simulink model "ZT_VehCtrl_18B_CAN"  (R2018b)
settings: Solver=FixedStepAuto  StartTime=0.0  StopTime=inf  FixedStep=0.005  RelTol=1e-3
InitFcn:
  | mbd_mpc_consistency_checks(bdroot(gcs));
values from neighbouring files (symbols this model uses):
  BatoverTempTh = single(80)    [VCU_INIT.m]
  BRS_PwrValid = single(5)    [VCU_INIT.m]
  BRSEnSpdTh1 = single(10)    [VCU_INIT.m]
  BRSEnSpdTh2 = single(20)    [VCU_INIT.m]
  MCUTempAlarmTh = single (60)    [VCU_INIT.m]
  mps2kmh = single(3.6)    [VCU_INIT.m]
  MtrPwrFac = single(1/9550)    [VCU_INIT.m]
  MtrTempAlarmTh = single (50)    [VCU_INIT.m]
  Padle1Signal1_Th = [PadleSignal1_min,PadleSignal1_max]    [VCU_INIT.m]
  Padle1Signal2_Th = [PadleSignal2_min,PadleSignal2_max]    [VCU_INIT.m]
  PadleSignal1_max = 3.84    [VCU_INIT.m]
  PadleSignal1_min = 0.75    [VCU_INIT.m]
  PadleSignal2_max = 1.92    [VCU_INIT.m]
  PadleSignal2_min = 0.375    [VCU_INIT.m]
  PadleValid = 0.05    [VCU_INIT.m]
  PwrLimFactor = single(0.5)    [VCU_INIT.m]
  Ratio = single(1)    [VCU_INIT.m]
  rpm2mps = single(2*pi/60 * WhlRadius/Ratio)    [VCU_INIT.m]
  SOCLowTh = single(20)    [VCU_INIT.m]
  VehPwrBackwardMax = VehPwrMax * single(0.3)    [VCU_INIT.m]
  VehPwrMax = single(MtrPwrMax * 4)    [VCU_INIT.m]
  VehTrqBackwardMax = VehTrqMax * single(0.3)    [VCU_INIT.m]
  VehTrqMax = single(MtrTrqMax * Ratio *4)    [VCU_INIT.m]
  WhlRadius = single(1)    [VCU_INIT.m]
undefined symbols (not defined in the file or in its folder): Delay_Charge, Delay_Discharge, fifo_0_vect, fifo_1_vect, LQFP, pts1_fifo_0_vect, pts1_fifo_1_vect, pts2_fifo_0_vect, pts2_fifo_1_vect, pts3_fifo_0_vect, pts3_fifo_1_vect, pts4_fifo_0_vect, pts4_fifo_1_vect
libraries: mbd_mpc574x_ec_toolbox x157, canmsglib x74, simulink x38
(part 4 of 12)

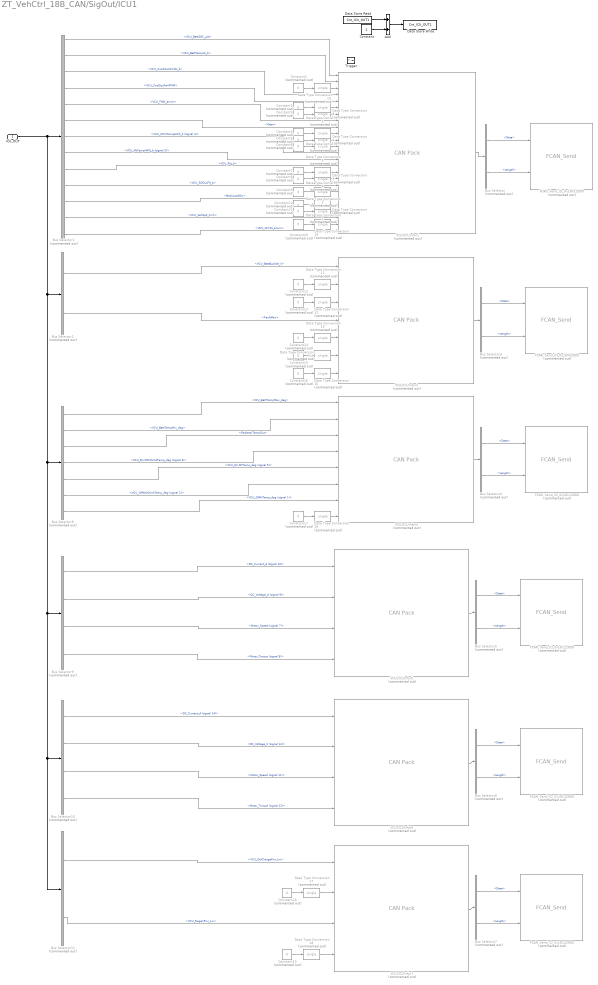
== system ZT_VehCtrl_18B_CAN/SigOut/ICU1  ==
  "ICU_OUT " : Inport
  Trigger : TriggerPort  VariantControl=Variant  PortDimensions=1
  Add : Sum
  Bus Selector{,3..7} (6 alike) : BusSelector  Commented=on  OutputSignals=Data,Length
  Bus Selector1 : BusSelector  Commented=on  OutputSignals=BMS.VCU_BattSOC_pct,BMS.VCU_BattTempHi_b,TMS.VCU_CoolFanWrkIdc_b,TMS.VCU_CoolSysFanPWM,Fault.VCU_FltSt_enum,Gear,MCU.VCU_MCUTempHiFlt_b (signal 4),MCU.VCU_MtTempHiFlt_b (signal 3),signal6.VCU_Pst_b,BMS.VCU_SOCLoFlt_b,signal6.BodyLoadSw,VCU_VehSpd_kmh,VCU_WrkSt_enum
  Bus Selector10 : BusSelector  Commented=on  OutputSignals=MCU.DC_Current_A (signal 14),MCU.DC_Voltage_V (signal 13),MCU.Motor_Speed (signal 11),MCU.Motor_Torque (signal 12)
  Bus Selector11 : BusSelector  Commented=on  OutputSignals=BMS.VCU_DisChargePwr_kw,BMS.VCU_RegenPwr_kw
  Bus Selector2 : BusSelector  Commented=on  OutputSignals=BMS.VCU_BattBusVolt_V,Fault.FaultMax
  Bus Selector8 : BusSelector  Commented=on  OutputSignals=BMS.VCU_BattTempMax_deg,BMS.VCU_BattTempMin_deg,signal6.RadiatorTempOut,MCU.VCU_DrvMtCtlUnitTemp_deg (signal 6),MCU.VCU_DrvMtTemp_deg (signal 5),MCU.VCU_OilMtCtlUnitTemp_deg (signal 2),MCU.VCU_OilMtTemp_deg (signal 1)
  Bus Selector9 : BusSelector  Commented=on  OutputSignals=MCU.DC_Current_A (signal 10),MCU.DC_Voltage_A (signal 9),MCU.Motor_Speed (signal 7),MCU.Motor_Torque (signal 8)
  Constant : Constant  OutDataTypeStr=uint8
  Constant{1..20} (20 alike) : Constant  Commented=on  Value=0  OutDataTypeStr=single
  Data Store Read : DataStoreRead  DataStoreName=Cnt_ICU_OUT1
  Data Store Write : DataStoreWrite  DataStoreName=Cnt_ICU_OUT1
  Data Type Conversion{,1..19} (20 alike) : DataTypeConversion  Commented=on  OutDataTypeStr=single
  FCAN_Send_ID_0x180128D0 : mbd_mpc574x_ec_toolbox/Communication Blocks/CAN Blocks/FCAN_Send  Priority=2  Commented=on  can_instance=0  can_mode=Non-blocking  can_timeout_ms=0  can_mb_idx=16  can_extended_id=on  can_is_remote=off  can_id=180128D0  show_adv_opts=off  can_fd_enable=off  can_enable_brs=off  can_fd_padding=0
      settings: SourceProductName=NXP Model-Based Design Toolbox for MPC57xx MCUs
  FCAN_Send_ID_0x180328D0 : mbd_mpc574x_ec_toolbox/Communication Blocks/CAN Blocks/FCAN_Send  Priority=2  Commented=on  can_instance=0  can_mode=Non-blocking  can_timeout_ms=0  can_mb_idx=18  can_extended_id=on  can_is_remote=off  can_id=180328D0  show_adv_opts=off  can_fd_enable=off  can_enable_brs=off  can_fd_padding=0
      settings: SourceProductName=NXP Model-Based Design Toolbox for MPC57xx MCUs
  FCAN_Send_ID_0x181128D0 : mbd_mpc574x_ec_toolbox/Communication Blocks/CAN Blocks/FCAN_Send  Priority=2  Commented=on  can_instance=0  can_mode=Non-blocking  can_timeout_ms=0  can_mb_idx=19  can_extended_id=on  can_is_remote=off  can_id=181128D0  show_adv_opts=off  can_fd_enable=off  can_enable_brs=off  can_fd_padding=0
      settings: SourceProductName=NXP Model-Based Design Toolbox for MPC57xx MCUs
  FCAN_Send_ID_0x181228D0 : mbd_mpc574x_ec_toolbox/Communication Blocks/CAN Blocks/FCAN_Send  Priority=2  Commented=on  can_instance=0  can_mode=Non-blocking  can_timeout_ms=0  can_mb_idx=20  can_extended_id=on  can_is_remote=off  can_id=181228D0  show_adv_opts=off  can_fd_enable=off  can_enable_brs=off  can_fd_padding=0
      settings: SourceProductName=NXP Model-Based Design Toolbox for MPC57xx MCUs
  FCAN_Send_ID_0x181328D0 : mbd_mpc574x_ec_toolbox/Communication Blocks/CAN Blocks/FCAN_Send  Priority=2  Commented=on  can_instance=0  can_mode=Non-blocking  can_timeout_ms=0  can_mb_idx=21  can_extended_id=on  can_is_remote=off  can_id=181328D0  show_adv_opts=off  can_fd_enable=off  can_enable_brs=off  can_fd_padding=0
      settings: SourceProductName=NXP Model-Based Design Toolbox for MPC57xx MCUs
  FCAN_Send_ID_0x181428D0 : mbd_mpc574x_ec_toolbox/Communication Blocks/CAN Blocks/FCAN_Send  Priority=2  Commented=on  can_instance=0  can_mode=Non-blocking  can_timeout_ms=0  can_mb_idx=22  can_extended_id=on  can_is_remote=off  can_id=181428D0  show_adv_opts=off  can_fd_enable=off  can_enable_brs=off  can_fd_padding=0
      settings: SourceProductName=NXP Model-Based Design Toolbox for MPC57xx MCUs
  VCU2ICUInfor1 : canmsglib/CAN Pack  Commented=on  CANdbFile=D:\VCU\VCU_SL_ZhengZhou\ZT2\模型与接口\CAN_DBC\整车CANA_GBK.dbc  MsgList=(none)  MsgName=VCU2ICUInfor1  MsgIDType=Extended (29-bit identifier)  MsgIdentifier=402729168  MsgLength=8  SignalInfo=VCU_BattSOC_pct$16$8$1$2$1$0$1$0$0$100$#VCU_BattTempHi_b$32$1$1$2$1$0$1$0$0$1$#VCU_BrakeFlt_b$39$1$1$2$1$0$1$0$0$1$#VCU_CoolFanWrkIdc_b$44$1$1$2$1$0$1$0$0$1$#VCU_CoolSysFanPWM$56$8$1$2$1$0$1$0$0$100$#VCU_CoolSysFltIdc_b$43$1$1$2$1$0$1$0$0$1$#VCU_EmrPumpSt_enum$5$2$1$2$1$0$1$0$0$3$#VCU_FltSt_enum$6$1$1$2$1$0$1$0$0$1$#VCU_GearSt_enum$24$8$1$2$1$0$1$0$0$5$#VCU_HeadLight_b$46$1$1$2$1$0$1$0$0$1$#VCU_HydSysFlt_b$33$1$1$2$1$0$1$0$0$1$#VCU_LShift_b$3$1$1$2$1$0$1$0$0$1$#VCU_MCUTempHiFlt_b$35$1$1$2$1$0$1$0$0$1$#VCU_MtTempHiFlt_b$36$1$1$2$1$0$1$0$0$1$#VCU_Pst_b$0$1$1$2$1$0$1$0$0$1$#VCU_RShift_b$2$1$1$2$1$0$1$0$0$1$#VCU_RearLight_b$45$1$1$2$1$0$1$0$0$1$#VCU_SOCLoFlt_b$1$1$1$2$1$0$1$0$0$1$#VCU_SysWorkStCode_num$48$8$1$2$1$0$1$0$0$255$#VCU_TopWrkSt_b$38$1$1$2$1$0$1$0$0$1$#VCU_VehACharge_b$34$1$1$2$1$0$1$0$0$1$#VCU_VehDCharge_b$37$1$1$2$1$0$1$0$0$1$#VCU_VehSpd_kmh$8$8$1$2$1$0$1$0$0$255$#VCU_WatPumpOpenSt_b$47$1$1$2$1$0$1$0$0$1$#VCU_WrkSt_enum$7$1$1$2$1$0$1$0$0$1$#  NSignals=25  StartBits=str2num('[int32(16);int32(32);int32(39);int32(44);int32(56);int32(43);int32(5);int32(6);int32(24);int32(46);int32(33);int32(3);int32(35);int32(36);int32(0);int32(2);int32(45);int32(1);int32(48);int32(38);int32(34);int32(37);int32(8);int32(47);int32(7)]')  SignalSizes=str2num('[int32(8);int32(1);int32(1);int32(1);int32(8);int32(1);int32(2);int32(1);int32(8);int32(1);int32(1);int32(1);int32(1);int32(1);int32(1);int32(1);int32(1);int32(1);int32(8);int32(1);int32(1);int32(1);int32(8);int32(1);int32(1)]')  ByteOrders=str2num('[int32(1);int32(1);int32(1);int32(1);int32(1);int32(1);int32(1);int32(1);int32(1);int32(1);int32(1);int32(1);int32(1);int32(1);int32(1);int32(1);int32(1);int32(1);int32(1);int32(1);int32(1);int32(1);int32(1);int32(1);int32(1)]')  DataTypes=str2num('[int32(2);int32(2);int32(2);int32(2);int32(2);int32(2);int32(2);int32(2);int32(2);int32(2);int32(2);int32(2);int32(2);int32(2);int32(2);int32(2);int32(2);int32(2);int32(2);int32(2);int32(2);int32(2);int32(2);int32(2);int32(2)]')  MultiplexTypes=str2num('[int32(1);int32(1);int32(1);int32(1);int32(1);int32(1);int32(1);int32(1);int32(1);int32(1);int32(1);int32(1);int32(1);int32(1);int32(1);int32(1);int32(1);int32(1);int32(1);int32(1);int32(1);int32(1);int32(1);int32(1);int32(1)]')  MultiplexValues=str2num('[double(0);double(0);double(0);double(0);double(0);double(0);double(0);double(0);double(0);double(0);double(0);double(0);double(0);double(0);double(0);double(0);double(0);double(0);double(0);double(0);double(0);double(0);double(0);double(0);double(0)]')  Factors=str2num('[double(1);double(1);double(1);double(1);double(1);double(1);double(1);double(1);double(1);double(1);double(1);double(1);double(1);double(1);double(1);double(1);double(1);double(1);double(1);double(1);double(1);double(1);double(1);double(1);double(1)]')  Offsets=str2num('[double(0);double(0);double(0);double(0);double(0);double(0);double(0);double(0);double(0);double(0);double(0);double(0);double(0);double(0);double(0);double(0);double(0);double(0);double(0);double(0);double(0);double(0);double(0);double(0);double(0)]')  Minimums=str2num('[double(0);double(0);double(0);double(0);double(0);double(0);double(0);double(0);double(0);double(0);double(0);double(0);double(0);double(0);double(0);double(0);double(0);double(0);double(0);double(0);double(0);double(0);double(0);double(0);double(0)]')  Maximums=str2num('[double(100);double(1);double(1);double(1);double(100);double(1);double(3);double(1);double(5);double(1);double(1);double(1);double(1);double(1);double(1);double(1);double(1);double(1);double(255);double(1);double(1);double(1);double(255);double(1);double(1)]')  Remote=off  ApplyMinMax=off  BusOutput=on
      settings: SourceProductName=Simulink Real-Time  SourceProductBaseCode=XP  DataFormat=CANdb specified signals
  VCU2ICUInfor3 : canmsglib/CAN Pack  Commented=on  CANdbFile=D:\VCU\VCU_SL_ZhengZhou\ZT2\模型与接口\CAN_DBC\整车CANA_GBK.dbc  MsgList=(none)  MsgName=VCU2ICUInfor3  MsgIDType=Extended (29-bit identifier)  MsgIdentifier=402860240  MsgLength=8  SignalInfo=VCU_BattBusVolt_V$48$16$1$2$1$0$1.000000e-01$0$0$6.553500e+03$#VCU_EVFltCode1_num$24$8$1$2$1$0$1$0$0$255$#VCU_EVFltCode2_num$32$8$1$2$1$0$1$0$0$255$#VCU_EVFltLvlMax_num$40$8$1$2$1$0$1$0$0$3$#VCU_HistFltCode1_num$0$8$1$2$1$0$1$0$0$255$#VCU_HistFltCode2_num$8$8$1$2$1$0$1$0$0$255$#VCU_HistFltCode3_num$16$8$1$2$1$0$1$0$0$255$#  NSignals=7  StartBits=str2num('[int32(48);int32(24);int32(32);int32(40);int32(0);int32(8);int32(16)]')  SignalSizes=str2num('[int32(16);int32(8);int32(8);int32(8);int32(8);int32(8);int32(8)]')  ByteOrders=str2num('[int32(1);int32(1);int32(1);int32(1);int32(1);int32(1);int32(1)]')  DataTypes=str2num('[int32(2);int32(2);int32(2);int32(2);int32(2);int32(2);int32(2)]')  MultiplexTypes=str2num('[int32(1);int32(1);int32(1);int32(1);int32(1);int32(1);int32(1)]')  MultiplexValues=str2num('[double(0);double(0);double(0);double(0);double(0);double(0);double(0)]')  Factors=str2num('[double(1.000000e-01);double(1);double(1);double(1);double(1);double(1);double(1)]')  Offsets=str2num('[double(0);double(0);double(0);double(0);double(0);double(0);double(0)]')  Minimums=str2num('[double(0);double(0);double(0);double(0);double(0);double(0);double(0)]')  Maximums=str2num('[double(6.553500e+03);double(255);double(255);double(3);double(255);double(255);double(255)]')  Remote=off  ApplyMinMax=off  BusOutput=on
      settings: SourceProductName=Simulink Real-Time  SourceProductBaseCode=XP  DataFormat=CANdb specified signals
  VCU2ICUInfor4 : canmsglib/CAN Pack  Commented=on  CANdbFile=D:\VCU\VCU_SL_ZhengZhou\ZT2\模型与接口\CAN_DBC\整车CANA_GBK.dbc  MsgList=(none)  MsgName=VCU2ICUInfor4  MsgIDType=Extended (29-bit identifier)  MsgIdentifier=403777744  MsgLength=8  SignalInfo=VCU_BattTempMax_deg$48$8$1$1$1$0$1$-40$-40$215$#VCU_BattTempMin_deg$40$8$1$1$1$0$1$-40$-40$215$#VCU_CoolWaterTemp_deg$16$8$1$1$1$0$1$-40$-40$215$#VCU_DrvMtCtlUnitTemp_deg$32$8$1$1$1$0$1$-40$-40$215$#VCU_DrvMtTemp_deg$24$8$1$1$1$0$1$-40$-40$215$#VCU_OilMtCtlUnitTemp_deg$8$8$1$1$1$0$1$-40$-40$215$#VCU_OilMtTemp_deg$0$8$1$1$1$0$1$-40$-40$215$#VCU_RemindInfor_num$56$8$1$2$1$0$1$0$-Inf$Inf$#  NSignals=8  StartBits=str2num('[int32(48);int32(40);int32(16);int32(32);int32(24);int32(8);int32(0);int32(56)]')  SignalSizes=str2num('[int32(8);int32(8);int32(8);int32(8);int32(8);int32(8);int32(8);int32(8)]')  ByteOrders=str2num('[int32(1);int32(1);int32(1);int32(1);int32(1);int32(1);int32(1);int32(1)]')  DataTypes=str2num('[int32(1);int32(1);int32(1);int32(1);int32(1);int32(1);int32(1);int32(2)]')  MultiplexTypes=str2num('[int32(1);int32(1);int32(1);int32(1);int32(1);int32(1);int32(1);int32(1)]')  MultiplexValues=str2num('[double(0);double(0);double(0);double(0);double(0);double(0);double(0);double(0)]')  Factors=str2num('[double(1);double(1);double(1);double(1);double(1);double(1);double(1);double(1)]')  Offsets=str2num('[double(-40);double(-40);double(-40);double(-40);double(-40);double(-40);double(-40);double(0)]')  Minimums=str2num('[double(-40);double(-40);double(-40);double(-40);double(-40);double(-40);double(-40);double(-Inf)]')  Maximums=str2num('[double(215);double(215);double(215);double(215);double(215);double(215);double(215);double(Inf)]')  Remote=off  ApplyMinMax=off  BusOutput=on
      settings: SourceProductName=Simulink Real-Time  SourceProductBaseCode=XP  DataFormat=CANdb specified signals
  VCU2ICUInfor5 : canmsglib/CAN Pack  Commented=on  CANdbFile=D:\VCU\VCU_SL_ZhengZhou\ZT2\模型与接口\CAN_DBC\整车CANA_GBK.dbc  MsgList=(none)  MsgName=VCU2ICUInfor5  MsgIDType=Extended (29-bit identifier)  MsgIdentifier=403843280  MsgLength=8  SignalInfo=VCU_DrvMCUBusCurr_A$48$16$1$1$1$0$1$-1000$-1000$35535$#VCU_DrvMCUBusVolt_V$32$16$1$2$1$0$1$0$0$65535$#VCU_DrvMtSpd_rpm$0$16$1$1$1$0$1$-30000$-30000$35535$#VCU_DrvMtTrq_Nm$16$16$1$2$1$0$1$0$0$65535$#  NSignals=4  StartBits=str2num('[int32(48);int32(32);int32(0);int32(16)]')  SignalSizes=str2num('[int32(16);int32(16);int32(16);int32(16)]')  ByteOrders=str2num('[int32(1);int32(1);int32(1);int32(1)]')  DataTypes=str2num('[int32(1);int32(2);int32(1);int32(2)]')  MultiplexTypes=str2num('[int32(1);int32(1);int32(1);int32(1)]')  MultiplexValues=str2num('[double(0);double(0);double(0);double(0)]')  Factors=str2num('[double(1);double(1);double(1);double(1)]')  Offsets=str2num('[double(-1000);double(0);double(-30000);double(0)]')  Minimums=str2num('[double(-1000);double(0);double(-30000);double(0)]')  Maximums=str2num('[double(35535);double(65535);double(35535);double(65535)]')  Remote=off  ApplyMinMax=off  BusOutput=on
      settings: SourceProductName=Simulink Real-Time  SourceProductBaseCode=XP  DataFormat=CANdb specified signals
  VCU2ICUInfor6 : canmsglib/CAN Pack  Commented=on  CANdbFile=D:\VCU\VCU_SL_ZhengZhou\ZT2\模型与接口\CAN_DBC\整车CANA_GBK.dbc  MsgList=(none)  MsgName=VCU2ICUInfor6  MsgIDType=Extended (29-bit identifier)  MsgIdentifier=403908816  MsgLength=8  SignalInfo=VCU_OilMCUBusCurr_A$48$16$1$1$1$0$1$-1000$-1000$35535$#VCU_OilMCUBusVolt_V$32$16$1$2$1$0$1$0$0$65535$#VCU_OilMtSpd_rpm$0$16$1$2$1$0$1$0$0$65535$#VCU_OilMtTrq_Nm$16$16$1$2$1$0$1$0$0$65535$#  NSignals=4  StartBits=str2num('[int32(48);int32(32);int32(0);int32(16)]')  SignalSizes=str2num('[int32(16);int32(16);int32(16);int32(16)]')  ByteOrders=str2num('[int32(1);int32(1);int32(1);int32(1)]')  DataTypes=str2num('[int32(1);int32(2);int32(2);int32(2)]')  MultiplexTypes=str2num('[int32(1);int32(1);int32(1);int32(1)]')  MultiplexValues=str2num('[double(0);double(0);double(0);double(0)]')  Factors=str2num('[double(1);double(1);double(1);double(1)]')  Offsets=str2num('[double(-1000);double(0);double(0);double(0)]')  Minimums=str2num('[double(-1000);double(0);double(0);double(0)]')  Maximums=str2num('[double(35535);double(65535);double(65535);double(65535)]')  Remote=off  ApplyMinMax=off  BusOutput=on
      settings: SourceProductName=Simulink Real-Time  SourceProductBaseCode=XP  DataFormat=CANdb specified signals
  VCU2ICUInfor7 : canmsglib/CAN Pack  Commented=on  CANdbFile=D:\VCU\VCU_SL_ZhengZhou\ZT2\模型与接口\CAN_DBC\整车CANA_GBK.dbc  MsgList=(none)  MsgName=VCU2ICUInfor7  MsgIDType=Extended (29-bit identifier)  MsgIdentifier=403974352  MsgLength=8  SignalInfo=VCU_DisChargePwr_kw$0$16$1$2$1$0$1.000000e-01$0$0$10000$#VCU_RangeRemain_km$48$16$1$2$1$0$1$0$0$65535$#VCU_RegenPwr_kw$16$16$1$2$1$0$1.000000e-01$0$0$10000$#VCU_RunAllMile_km$32$16$1$2$1$0$1$0$0$65535$#  NSignals=4  StartBits=str2num('[int32(0);int32(48);int32(16);int32(32)]')  SignalSizes=str2num('[int32(16);int32(16);int32(16);int32(16)]')  ByteOrders=str2num('[int32(1);int32(1);int32(1);int32(1)]')  DataTypes=str2num('[int32(2);int32(2);int32(2);int32(2)]')  MultiplexTypes=str2num('[int32(1);int32(1);int32(1);int32(1)]')  MultiplexValues=str2num('[double(0);double(0);double(0);double(0)]')  Factors=str2num('[double(1.000000e-01);double(1);double(1.000000e-01);double(1)]')  Offsets=str2num('[double(0);double(0);double(0);double(0)]')  Minimums=str2num('[double(0);double(0);double(0);double(0)]')  Maximums=str2num('[double(10000);double(65535);double(10000);double(65535)]')  Remote=off  ApplyMinMax=off  BusOutput=on
      settings: SourceProductName=Simulink Real-Time  SourceProductBaseCode=XP  DataFormat=CANdb specified signals
  wires:
  VCU2ICUInfor1/1 -> Bus Selector/1
  Bus Selector/1 -> FCAN_Send_ID_0x180128D0/1  "<Data>"
  Bus Selector/2 -> FCAN_Send_ID_0x180128D0/2  "<Length>"
  VCU2ICUInfor3/1 -> Bus Selector3/1
  Bus Selector3/1 -> FCAN_Send_ID_0x180328D0/1  "<Data>"
  Bus Selector3/2 -> FCAN_Send_ID_0x180328D0/2  "<Length>"
  Bus Selector4/2 -> FCAN_Send_ID_0x181128D0/2  "<Length>"
  Bus Selector4/1 -> FCAN_Send_ID_0x181128D0/1  "<Data>"
  VCU2ICUInfor4/1 -> Bus Selector4/1
  VCU2ICUInfor5/1 -> Bus Selector5/1
  Bus Selector5/1 -> FCAN_Send_ID_0x181228D0/1  "<Data>"
  Bus Selector5/2 -> FCAN_Send_ID_0x181228D0/2  "<Length>"
  Bus Selector6/2 -> FCAN_Send_ID_0x181328D0/2  "<Length>"
  Bus Selector6/1 -> FCAN_Send_ID_0x181328D0/1  "<Data>"
  VCU2ICUInfor6/1 -> Bus Selector6/1
  VCU2ICUInfor7/1 -> Bus Selector7/1
  Bus Selector7/1 -> FCAN_Send_ID_0x181428D0/1  "<Data>"
  Bus Selector7/2 -> FCAN_Send_ID_0x181428D0/2  "<Length>"
  "ICU_OUT "/1 -> Bus Selector11/1, Bus Selector10/1, Bus Selector9/1, Bus Selector8/1, Bus Selector2/1, Bus Selector1/1
  Add/1 -> Data Store Write/1
  Data Store Read/1 -> Add/1
  Constant/1 -> Add/2
  Bus Selector1/1 -> VCU2ICUInfor1/1  "<VCU_BattSOC_pct>"
  Bus Selector1/2 -> VCU2ICUInfor1/2  "<VCU_BattTempHi_b>"
  Bus Selector1/3 -> VCU2ICUInfor1/4  "<VCU_CoolFanWrkIdc_b>"
  Bus Selector1/4 -> VCU2ICUInfor1/5  "<VCU_CoolSysFanPWM>"
  Constant1/1 -> Data Type Conversion10/1
  Bus Selector1/5 -> VCU2ICUInfor1/8  "<VCU_FltSt_enum>"
  Bus Selector1/6 -> VCU2ICUInfor1/9  "<Gear>"
  Bus Selector1/7 -> VCU2ICUInfor1/13  "<VCU_MCUTempHiFlt_b (signal 4)>"
  Bus Selector1/8 -> VCU2ICUInfor1/14  "<VCU_MtTempHiFlt_b (signal 3)>"
  Bus Selector1/9 -> VCU2ICUInfor1/15  "<VCU_Pst_b>"
  Bus Selector1/10 -> VCU2ICUInfor1/18  "<VCU_SOCLoFlt_b>"
  Bus Selector1/11 -> VCU2ICUInfor1/20  "<BodyLoadSw>"
  Bus Selector1/12 -> VCU2ICUInfor1/23  "<VCU_VehSpd_kmh>"
  Bus Selector1/13 -> VCU2ICUInfor1/25  "<VCU_WrkSt_enum>"
  Constant2/1 -> Data Type Conversion9/1
  Constant3/1 -> Data Type Conversion8/1
  Constant4/1 -> Data Type Conversion7/1
  Constant5/1 -> Data Type Conversion6/1
  Constant6/1 -> Data Type Conversion5/1
  Constant7/1 -> Data Type Conversion4/1
  Constant8/1 -> Data Type Conversion3/1
  Constant9/1 -> Data Type Conversion2/1
  Constant10/1 -> Data Type Conversion1/1
  Constant11/1 -> Data Type Conversion/1
  Bus Selector2/1 -> VCU2ICUInfor3/1  "<VCU_BattBusVolt_V>"
  Bus Selector2/2 -> VCU2ICUInfor3/4  "<FaultMax>"
  Data Type Conversion/1 -> VCU2ICUInfor1/22
  Data Type Conversion1/1 -> VCU2ICUInfor1/21
  Data Type Conversion2/1 -> VCU2ICUInfor1/19
  Data Type Conversion3/1 -> VCU2ICUInfor1/17
  Data Type Conversion4/1 -> VCU2ICUInfor1/16
  Data Type Conversion5/1 -> VCU2ICUInfor1/12
  Data Type Conversion6/1 -> VCU2ICUInfor1/11
  Data Type Conversion7/1 -> VCU2ICUInfor1/10
  Data Type Conversion8/1 -> VCU2ICUInfor1/7
  Data Type Conversion9/1 -> VCU2ICUInfor1/6
  Data Type Conversion10/1 -> VCU2ICUInfor1/3
  Constant12/1 -> Data Type Conversion11/1
  Data Type Conversion11/1 -> VCU2ICUInfor3/2
  Constant13/1 -> Data Type Conversion12/1
  Data Type Conversion12/1 -> VCU2ICUInfor3/3
  Constant14/1 -> Data Type Conversion13/1
  Data Type Conversion13/1 -> VCU2ICUInfor3/5
  Constant15/1 -> Data Type Conversion14/1
  Data Type Conversion14/1 -> VCU2ICUInfor3/6
  Constant16/1 -> Data Type Conversion15/1
  Data Type Conversion15/1 -> VCU2ICUInfor3/7
  Bus Selector8/1 -> VCU2ICUInfor4/1  "<VCU_BattTempMax_deg>"
  Bus Selector8/2 -> VCU2ICUInfor4/2  "<VCU_BattTempMin_deg>"
  Bus Selector8/3 -> VCU2ICUInfor4/3  "<RadiatorTempOut>"
  Bus Selector8/4 -> VCU2ICUInfor4/4  "<VCU_DrvMtCtlUnitTemp_deg (signal 6)>"
  Bus Selector8/5 -> VCU2ICUInfor4/5  "<VCU_DrvMtTemp_deg (signal 5)>"
  Bus Selector8/6 -> VCU2ICUInfor4/6  "<VCU_OilMtCtlUnitTemp_deg (signal 2)>"
  Bus Selector8/7 -> VCU2ICUInfor4/7  "<VCU_OilMtTemp_deg (signal 1)>"
  Constant17/1 -> Data Type Conversion16/1
  Data Type Conversion16/1 -> VCU2ICUInfor4/8
  Bus Selector9/1 -> VCU2ICUInfor5/1  "<DC_Current_A (signal 10)>"
  Bus Selector9/2 -> VCU2ICUInfor5/2  "<DC_Voltage_A (signal 9)>"
  Bus Selector9/3 -> VCU2ICUInfor5/3  "<Motor_Speed (signal 7)>"
  Bus Selector9/4 -> VCU2ICUInfor5/4  "<Motor_Torque (signal 8)>"
  Bus Selector10/1 -> VCU2ICUInfor6/1  "<DC_Current_A (signal 14)>"
  Bus Selector10/2 -> VCU2ICUInfor6/2  "<DC_Voltage_V (signal 13)>"
  Bus Selector10/3 -> VCU2ICUInfor6/3  "<Motor_Speed (signal 11)>"
  Bus Selector10/4 -> VCU2ICUInfor6/4  "<Motor_Torque (signal 12)>"
  Bus Selector11/1 -> VCU2ICUInfor7/1  "<VCU_DisChargePwr_kw>"
  Bus Selector11/2 -> VCU2ICUInfor7/3  "<VCU_RegenPwr_kw>"
  Data Type Conversion17/1 -> VCU2ICUInfor7/2
  Constant18/1 -> Data Type Conversion17/1
  Constant19/1 -> Data Type Conversion18/1
  Data Type Conversion18/1 -> VCU2ICUInfor7/4
  Data Type Conversion19/1 -> VCU2ICUInfor1/24
  Constant20/1 -> Data Type Conversion19/1

== system ZT_VehCtrl_18B_CAN/SigOut/ICU2 ==
  "ICU_OUT " : Inport
  Trigger : TriggerPort  VariantControl=Variant  PortDimensions=1
  Add : Sum
  Bus Selector : BusSelector  Commented=on  OutputSignals=Data,Length
  Bus Selector2 : BusSelector  Commented=on  OutputSignals=signal6.AccPadle,BMS.VCU_BattBusCurr_A
  Constant : Constant  OutDataTypeStr=uint8
  Constant{1..4} (4 alike) : Constant  Commented=on  Value=0
  Data Store Read : DataStoreRead  DataStoreName=Cnt_ICU_OUT2
  Data Store Write : DataStoreWrite  DataStoreName=Cnt_ICU_OUT2
  Data Type Conversion{,1..5} (6 alike) : DataTypeConversion  Commented=on  OutDataTypeStr=single
  FCAN_Send_ID_0x180228D0 : mbd_mpc574x_ec_toolbox/Communication Blocks/CAN Blocks/FCAN_Send  Priority=2  Commented=on  can_instance=0  can_mode=Non-blocking  can_timeout_ms=0  can_mb_idx=17  can_extended_id=on  can_is_remote=off  can_id=180228D0  show_adv_opts=off  can_fd_enable=off  can_enable_brs=off  can_fd_padding=0
      settings: SourceProductName=NXP Model-Based Design Toolbox for MPC57xx MCUs
  VCU2ICUInfor2 : canmsglib/CAN Pack  Commented=on  CANdbFile=D:\VCU\VCU_SL_ZhengZhou\ZT2\模型与接口\CAN_DBC\整车CANA_GBK.dbc  MsgList=(none)  MsgName=VCU2ICUInfor2  MsgIDType=Extended (29-bit identifier)  MsgIdentifier=402794704  MsgLength=8  SignalInfo=VCU_AccPedSt_pct$24$8$1$2$1$0$1$0$0$100$#VCU_BattBusCurr_A$8$16$1$1$1$0$1.000000e-01$-1000$-1000$-1000$#VCU_BrakePedSt_pct$32$8$1$2$1$0$1$0$0$100$#VCU_SwVersion_num$0$8$1$2$1$0$1.000000e-01$0$0$255$#VCU_WrkTimeAll_h$40$16$1$2$1$0$1$0$0$65535$#VCU_WrkTimeAll_min$56$8$1$2$1$0$1$0$0$255$#  NSignals=6  StartBits=str2num('[int32(24);int32(8);int32(32);int32(0);int32(40);int32(56)]')  SignalSizes=str2num('[int32(8);int32(16);int32(8);int32(8);int32(16);int32(8)]')  ByteOrders=str2num('[int32(1);int32(1);int32(1);int32(1);int32(1);int32(1)]')  DataTypes=str2num('[int32(2);int32(1);int32(2);int32(2);int32(2);int32(2)]')  MultiplexTypes=str2num('[int32(1);int32(1);int32(1);int32(1);int32(1);int32(1)]')  MultiplexValues=str2num('[double(0);double(0);double(0);double(0);double(0);double(0)]')  Factors=str2num('[double(1);double(1.000000e-01);double(1);double(1.000000e-01);double(1);double(1)]')  Offsets=str2num('[double(0);double(-1000);double(0);double(0);double(0);double(0)]')  Minimums=str2num('[double(0);double(-1000);double(0);double(0);double(0);double(0)]')  Maximums=str2num('[double(100);double(-1000);double(100);double(255);double(65535);double(255)]')  Remote=off  ApplyMinMax=off  BusOutput=on
      settings: SourceProductName=Simulink Real-Time  SourceProductBaseCode=XP  DataFormat=CANdb specified signals
  wires:
  Bus Selector/2 -> FCAN_Send_ID_0x180228D0/2  "<Length>"
  Bus Selector/1 -> FCAN_Send_ID_0x180228D0/1  "<Data>"
  VCU2ICUInfor2/1 -> Bus Selector/1
  "ICU_OUT "/1 -> Bus Selector2/1
  Add/1 -> Data Store Write/1
  Data Store Read/1 -> Add/1
  Constant/1 -> Add/2
  Bus Selector2/1 -> Data Type Conversion/1  "<AccPadle>"
  Bus Selector2/2 -> Data Type Conversion1/1  "<VCU_BattBusCurr_A>"
  Data Type Conversion/1 -> VCU2ICUInfor2/1
  Data Type Conversion1/1 -> VCU2ICUInfor2/2
  Constant1/1 -> Data Type Conversion2/1
  Data Type Conversion2/1 -> VCU2ICUInfor2/3
  Constant2/1 -> Data Type Conversion3/1
  Data Type Conversion3/1 -> VCU2ICUInfor2/4
  Data Type Conversion4/1 -> VCU2ICUInfor2/5
  Constant3/1 -> Data Type Conversion4/1
  Constant4/1 -> Data Type Conversion5/1
  Data Type Conversion5/1 -> VCU2ICUInfor2/6

== system ZT_VehCtrl_18B_CAN/SigOut/ISG ==
  "ISG_OUT " : Inport
  Trigger : TriggerPort  VariantControl=Variant  PortDimensions=1
  Add : Sum
  Bus Selector : BusSelector  OutputSignals=Data,Length
  Constant : Constant  OutDataTypeStr=uint8
  Constant{1..10} (10 alike) : Constant  Value=0
  Data Store Read : DataStoreRead  DataStoreName=Cnt_ISG_OUT
  Data Store Write : DataStoreWrite  DataStoreName=Cnt_ISG_OUT
  FCAN_Send_ID_0xCFF06EF : mbd_mpc574x_ec_toolbox/Communication Blocks/CAN Blocks/FCAN_Send  Priority=2  can_instance=1  can_mode=Non-blocking  can_timeout_ms=0  can_mb_idx=54  can_extended_id=on  can_is_remote=off  can_id=CFF06EF  show_adv_opts=off  can_fd_enable=off  can_enable_brs=off  can_fd_padding=0
      settings: SourceProductName=NXP Model-Based Design Toolbox for MPC57xx MCUs
  ISG HCU Command : canmsglib/CAN Pack  CANdbFile=D:\VCU\VCU_SL_ZhengZhou\ZT2\模型与接口\CAN_DBC\动力CANB_GBK.dbc  MsgList=(none)  MsgName=ISG_HCU_Command  MsgIDType=Extended (29-bit identifier)  MsgIdentifier=218040047  MsgLength=8  SignalInfo=Control_Mode$2$2$1$2$1$0$1$0$-Inf$Inf$#Demand_Limit_High_Positive_Value$8$12$1$2$1$0$4$0$0$16384$#Demand_Limit_Low_Negative_Value$20$12$1$2$1$0$4$0$0$16384$#Demand_Speed$48$16$1$2$1$0$1$-15000$-15000$15000$#Demand_Torque$32$16$1$2$1$0$1$-5000$-5000$5000$#Fault_Reset$1$1$1$2$1$0$1$0$-Inf$Inf$#FootBrake$6$1$1$2$1$0$1$0$-Inf$Inf$#Gear$4$2$1$2$1$0$1$0$-Inf$Inf$#HandBrake$7$1$1$2$1$0$1$0$-Inf$Inf$#MCU_Enable$0$1$1$2$1$0$1$0$-Inf$Inf$#  NSignals=10  StartBits=str2num('[int32(2);int32(8);int32(20);int32(48);int32(32);int32(1);int32(6);int32(4);int32(7);int32(0)]')  SignalSizes=str2num('[int32(2);int32(12);int32(12);int32(16);int32(16);int32(1);int32(1);int32(2);int32(1);int32(1)]')  ByteOrders=str2num('[int32(1);int32(1);int32(1);int32(1);int32(1);int32(1);int32(1);int32(1);int32(1);int32(1)]')  DataTypes=str2num('[int32(2);int32(2);int32(2);int32(2);int32(2);int32(2);int32(2);int32(2);int32(2);int32(2)]')  MultiplexTypes=str2num('[int32(1);int32(1);int32(1);int32(1);int32(1);int32(1);int32(1);int32(1);int32(1);int32(1)]')  MultiplexValues=str2num('[double(0);double(0);double(0);double(0);double(0);double(0);double(0);double(0);double(0);double(0)]')  Factors=str2num('[double(1);double(4);double(4);double(1);double(1);double(1);double(1);double(1);double(1);double(1)]')  Offsets=str2num('[double(0);double(0);double(0);double(-15000);double(-5000);double(0);double(0);double(0);double(0);double(0)]')  Minimums=str2num('[double(-Inf);double(0);double(0);double(-15000);double(-5000);double(-Inf);double(-Inf);double(-Inf);double(-Inf);double(-Inf)]')  Maximums=str2num('[double(Inf);double(16384);double(16384);double(15000);double(5000);double(Inf);double(Inf);double(Inf);double(Inf);double(Inf)]')  Remote=off  ApplyMinMax=off  BusOutput=on
      settings: SourceProductName=Simulink Real-Time  SourceProductBaseCode=XP  DataFormat=CANdb specified signals
  Terminator : Terminator
  wires:
  ISG HCU Command/1 -> Bus Selector/1
  Bus Selector/2 -> FCAN_Send_ID_0xCFF06EF/2  "<Length>"
  Bus Selector/1 -> FCAN_Send_ID_0xCFF06EF/1  "<Data>"
  "ISG_OUT "/1 -> Terminator/1
  Constant1/1 -> ISG HCU Command/1
  Constant2/1 -> ISG HCU Command/2
  Constant3/1 -> ISG HCU Command/3
  Constant4/1 -> ISG HCU Command/4
  Constant5/1 -> ISG HCU Command/5
  Constant6/1 -> ISG HCU Command/6
  Constant7/1 -> ISG HCU Command/7
  Constant8/1 -> ISG HCU Command/8
  Constant9/1 -> ISG HCU Command/9
  Constant10/1 -> ISG HCU Command/10
  Add/1 -> Data Store Write/1
  Data Store Read/1 -> Add/1
  Constant/1 -> Add/2

== system ZT_VehCtrl_18B_CAN/SigOut/MCU1 ==
  "MCU_OUT " : Inport
  Trigger : TriggerPort  VariantControl=Variant  PortDimensions=1
  Add : Sum
  Bus Selector : BusSelector  OutputSignals=Data,Length
  Bus Selector1 : BusSelector  OutputSignals=signal1.VCU2OilMotor_ActiveDisCharge,Enable
  Constant : Constant  OutDataTypeStr=uint8
  Data Store Read : DataStoreRead  DataStoreName=Cnt_MCU1_OUT
  Data Store Write : DataStoreWrite  DataStoreName=Cnt_MCU1_OUT
  FCAN_Send_ID_0x0C31EFD0 : mbd_mpc574x_ec_toolbox/Communication Blocks/CAN Blocks/FCAN_Send  Priority=2  can_instance=1  can_mode=Non-blocking  can_timeout_ms=0  can_mb_idx=49  can_extended_id=on  can_is_remote=off  can_id=0C31EFD0  show_adv_opts=off  can_fd_enable=off  can_enable_brs=off  can_fd_padding=0
      settings: SourceProductName=NXP Model-Based Design Toolbox for MPC57xx MCUs
  VCU2MCU1 : canmsglib/CAN Pack  CANdbFile=D:\VCU\VCU_SL_ZhengZhou\ZT2\模型与接口\CAN_DBC\动力CANB_GBK.dbc  MsgList=(none)  MsgName=VCU2MCU1  MsgIDType=Extended (29-bit identifier)  MsgIdentifier=204599248  MsgLength=8  SignalInfo=VCU2OilMotor_ActiveDisCharge$5$1$1$2$1$0$1$0$0$1$#VCU2OilMotor_AntiSlipEn$4$1$1$2$1$0$1$0$0$1$#VCU2OilMotor_BusCurLimit$8$8$1$2$1$0$4$0$0$1000$#VCU2OilMotor_CtrlBusCounter$56$8$1$2$1$0$1$0$0$255$#VCU2OilMotor_CtrlMode$3$1$1$2$1$0$1$0$0$1$#VCU2OilMotor_En$0$1$1$2$1$0$1$0$0$1$#VCU2OilMotor_RegenVoltLimit$48$8$1$2$1$0$4$0$0$255$#VCU2OilMotor_TarSpd$16$16$1$2$1$0$2.500000e-01$0$0$1.638375e+04$#VCU2OilMotor_TarTrq$32$16$1$2$1$0$1.000000e-01$0$0$6.553500e+03$#VCU2OilMotor_WorkMode$1$2$1$2$1$0$1$0$0$3$#  NSignals=10  StartBits=str2num('[int32(5);int32(4);int32(8);int32(56);int32(3);int32(0);int32(48);int32(16);int32(32);int32(1)]')  SignalSizes=str2num('[int32(1);int32(1);int32(8);int32(8);int32(1);int32(1);int32(8);int32(16);int32(16);int32(2)]')  ByteOrders=str2num('[int32(1);int32(1);int32(1);int32(1);int32(1);int32(1);int32(1);int32(1);int32(1);int32(1)]')  DataTypes=str2num('[int32(2);int32(2);int32(2);int32(2);int32(2);int32(2);int32(2);int32(2);int32(2);int32(2)]')  MultiplexTypes=str2num('[int32(1);int32(1);int32(1);int32(1);int32(1);int32(1);int32(1);int32(1);int32(1);int32(1)]')  MultiplexValues=str2num('[double(0);double(0);double(0);double(0);double(0);double(0);double(0);double(0);double(0);double(0)]')  Factors=str2num('[double(1);double(1);double(4);double(1);double(1);double(1);double(4);double(2.500000e-01);double(1.000000e-01);double(1)]')  Offsets=str2num('[double(0);double(0);double(0);double(0);double(0);double(0);double(0);double(0);double(0);double(0)]')  Minimums=str2num('[double(0);double(0);double(0);double(0);double(0);double(0);double(0);double(0);double(0);double(0)]')  Maximums=str2num('[double(1);double(1);double(1000);double(255);double(1);double(1);double(255);double(1.638375e+04);double(6.553500e+03);double(3)]')  Remote=off  ApplyMinMax=off  BusOutput=on
      settings: SourceProductName=Simulink Real-Time  SourceProductBaseCode=XP  DataFormat=CANdb specified signals
  wires:
  VCU2MCU1/1 -> Bus Selector/1
  Bus Selector/2 -> FCAN_Send_ID_0x0C31EFD0/2  "<Length>"
  Bus Selector/1 -> FCAN_Send_ID_0x0C31EFD0/1  "<Data>"
  Add/1 -> Data Store Write/1
  Data Store Read/1 -> Add/1
  Constant/1 -> Add/2
  "MCU_OUT "/1 -> Bus Selector1/1
  Bus Selector1/2 -> VCU2MCU1/6  "<Enable>"
  Bus Selector1/1 -> VCU2MCU1/1  "<VCU2OilMotor_ActiveDisCharge>"

== system ZT_VehCtrl_18B_CAN/SigOut/MCU2 ==
  "MCU_OUT " : Inport
  Trigger : TriggerPort  VariantControl=Variant  PortDimensions=1
  Add : Sum
  Bus Selector1 : BusSelector  OutputSignals=Data,Length
  Constant : Constant  OutDataTypeStr=uint8
  Constant{11..20} (10 alike) : Constant  Value=0
  Data Store Read : DataStoreRead  DataStoreName=Cnt_MCU2_OUT
  Data Store Write : DataStoreWrite  DataStoreName=Cnt_MCU2_OUT
  FCAN_Send_ID_0x0C31F1D0 : mbd_mpc574x_ec_toolbox/Communication Blocks/CAN Blocks/FCAN_Send  Priority=2  can_instance=1  can_mode=Non-blocking  can_timeout_ms=0  can_mb_idx=50  can_extended_id=on  can_is_remote=off  can_id=0C31F1D0  show_adv_opts=off  can_fd_enable=off  can_enable_brs=off  can_fd_padding=0
      settings: SourceProductName=NXP Model-Based Design Toolbox for MPC57xx MCUs
  Terminator : Terminator
  VCU2MCU2 : canmsglib/CAN Pack  CANdbFile=D:\VCU\VCU_SL_ZhengZhou\ZT2\模型与接口\CAN_DBC\动力CANB_GBK.dbc  MsgList=(none)  MsgName=VCU2MCU2  MsgIDType=Extended (29-bit identifier)  MsgIdentifier=204599760  MsgLength=8  SignalInfo=VCU2DrvMotor_ActiveDisCharge$5$1$1$2$1$0$1$0$0$1$#VCU2DrvMotor_AntiSlipEn$4$1$1$2$1$0$1$0$0$1$#VCU2DrvMotor_BusCurLimit$8$8$1$2$1$0$4$0$0$1000$#VCU2DrvMotor_CtrlBusCounter$56$8$1$2$1$0$1$0$0$255$#VCU2DrvMotor_CtrlMode$3$1$1$2$1$0$1$0$0$1$#VCU2DrvMotor_En$0$1$1$2$1$0$1$0$0$1$#VCU2DrvMotor_RegenVoltLimit$48$8$1$2$1$0$4$0$0$255$#VCU2DrvMotor_TarSpd$16$16$1$2$1$0$2.500000e-01$0$0$1.638375e+04$#VCU2DrvMotor_TarTrq$32$16$1$2$1$0$1.000000e-01$0$0$6.553500e+03$#VCU2DrvMotor_WorkMode$1$2$1$2$1$0$1$0$0$3$#  NSignals=10  StartBits=str2num('[int32(5);int32(4);int32(8);int32(56);int32(3);int32(0);int32(48);int32(16);int32(32);int32(1)]')  SignalSizes=str2num('[int32(1);int32(1);int32(8);int32(8);int32(1);int32(1);int32(8);int32(16);int32(16);int32(2)]')  ByteOrders=str2num('[int32(1);int32(1);int32(1);int32(1);int32(1);int32(1);int32(1);int32(1);int32(1);int32(1)]')  DataTypes=str2num('[int32(2);int32(2);int32(2);int32(2);int32(2);int32(2);int32(2);int32(2);int32(2);int32(2)]')  MultiplexTypes=str2num('[int32(1);int32(1);int32(1);int32(1);int32(1);int32(1);int32(1);int32(1);int32(1);int32(1)]')  MultiplexValues=str2num('[double(0);double(0);double(0);double(0);double(0);double(0);double(0);double(0);double(0);double(0)]')  Factors=str2num('[double(1);double(1);double(4);double(1);double(1);double(1);double(4);double(2.500000e-01);double(1.000000e-01);double(1)]')  Offsets=str2num('[double(0);double(0);double(0);double(0);double(0);double(0);double(0);double(0);double(0);double(0)]')  Minimums=str2num('[double(0);double(0);double(0);double(0);double(0);double(0);double(0);double(0);double(0);double(0)]')  Maximums=str2num('[double(1);double(1);double(1000);double(255);double(1);double(1);double(255);double(1.638375e+04);double(6.553500e+03);double(3)]')  Remote=off  ApplyMinMax=off  BusOutput=on
      settings: SourceProductName=Simulink Real-Time  SourceProductBaseCode=XP  DataFormat=CANdb specified signals
  wires:
  Constant/1 -> Add/2
  Data Store Read/1 -> Add/1
  Add/1 -> Data Store Write/1
  Constant20/1 -> VCU2MCU2/10
  Constant19/1 -> VCU2MCU2/9
  Constant18/1 -> VCU2MCU2/8
  Constant17/1 -> VCU2MCU2/7
  Constant16/1 -> VCU2MCU2/6
  Constant15/1 -> VCU2MCU2/5
  Constant14/1 -> VCU2MCU2/4
  Constant13/1 -> VCU2MCU2/3
  Constant12/1 -> VCU2MCU2/2
  Constant11/1 -> VCU2MCU2/1
  "MCU_OUT "/1 -> Terminator/1
  VCU2MCU2/1 -> Bus Selector1/1
  Bus Selector1/2 -> FCAN_Send_ID_0x0C31F1D0/2  "<Length>"
  Bus Selector1/1 -> FCAN_Send_ID_0x0C31F1D0/1  "<Data>"

== system ZT_VehCtrl_18B_CAN/SigOut/PDU ==
  "PDU_OUT " : Inport
  Trigger : TriggerPort  VariantControl=Variant  PortDimensions=1
  Add : Sum
  Bus Selector : BusSelector  OutputSignals=Data,Length
  Bus Selector1 : BusSelector  Commented=on  OutputSignals=VCU_DCCpstRlyCtl,VCU_HghVtgCtl,VCU_ShrRlyCtl
  Constant : Constant  OutDataTypeStr=uint8
  Data Store Read : DataStoreRead  DataStoreName=Cnt_PDU_OUT
  Data Store Read1 : DataStoreRead  DataStoreName=Cnt_PDU_OUT
  Data Store Read5 : DataStoreRead  DataStoreName=VCU_ShrRlyCtl
  Data Store Read6 : DataStoreRead  DataStoreName=VCU_HVACRlyCtl
  Data Store Read7 : DataStoreRead  DataStoreName=VCU_PTCRlyCtl
  Data Store Read8 : DataStoreRead  DataStoreName=VCU_HghVtgCnt
  Data Store Read9 : DataStoreRead  DataStoreName=VCU_DCCpstRlyCtl
  Data Store Write : DataStoreWrite  DataStoreName=Cnt_PDU_OUT
  Data Type Conversion{,1..5} (6 alike) : DataTypeConversion  OutDataTypeStr=single
  FCAN_Send_ID_0x0CF2503B : mbd_mpc574x_ec_toolbox/Communication Blocks/CAN Blocks/FCAN_Send  Priority=2  can_instance=0  can_mode=Non-blocking  can_timeout_ms=0  can_mb_idx=52  can_extended_id=on  can_is_remote=off  can_id=0CF2503B  show_adv_opts=off  can_fd_enable=off  can_enable_brs=off  can_fd_padding=0
      settings: SourceProductName=NXP Model-Based Design Toolbox for MPC57xx MCUs
  VCU_PDU : canmsglib/CAN Pack  CANdbFile=D:\VCU\VCU_SL_ZhengZhou\ZT2\Module\CAN_DBC\动力CANB_GBK.dbc  MsgList=(none)  MsgName=VCU_PDU  MsgIDType=Extended (29-bit identifier)  MsgIdentifier=217206843  MsgLength=8  SignalInfo=VCU_DCCpstRlyCtl$40$2$1$2$1$0$1$0$-Inf$Inf$#VCU_HVACRlyCtl$6$2$1$2$1$0$1$0$-Inf$Inf$#VCU_HghVtgCtl$16$2$1$2$1$0$1$0$-Inf$Inf$#VCU_HrtBt$56$8$1$2$1$0$1$0$-Inf$Inf$#VCU_PTCRlyCtl$8$2$1$2$1$0$1$0$-Inf$Inf$#VCU_ShrRlyCtl$0$2$1$2$1$0$1$0$-Inf$Inf$#  NSignals=6  StartBits=str2num('[int32(40);int32(6);int32(16);int32(56);int32(8);int32(0)]')  SignalSizes=str2num('[int32(2);int32(2);int32(2);int32(8);int32(2);int32(2)]')  ByteOrders=str2num('[int32(1);int32(1);int32(1);int32(1);int32(1);int32(1)]')  DataTypes=str2num('[int32(2);int32(2);int32(2);int32(2);int32(2);int32(2)]')  MultiplexTypes=str2num('[int32(1);int32(1);int32(1);int32(1);int32(1);int32(1)]')  MultiplexValues=str2num('[double(0);double(0);double(0);double(0);double(0);double(0)]')  Factors=str2num('[double(1);double(1);double(1);double(1);double(1);double(1)]')  Offsets=str2num('[double(0);double(0);double(0);double(0);double(0);double(0)]')  Minimums=str2num('[double(-Inf);double(-Inf);double(-Inf);double(-Inf);double(-Inf);double(-Inf)]')  Maximums=str2num('[double(Inf);double(Inf);double(Inf);double(Inf);double(Inf);double(Inf)]')  Remote=off  ApplyMinMax=off  BusOutput=on
      settings: SourceProductName=Simulink Real-Time  SourceProductBaseCode=XP  DataFormat=CANdb specified signals
  wires:
  Bus Selector/1 -> FCAN_Send_ID_0x0CF2503B/1  "<Data>"
  Bus Selector/2 -> FCAN_Send_ID_0x0CF2503B/2  "<Length>"
  VCU_PDU/1 -> Bus Selector/1
  Add/1 -> Data Store Write/1
  Data Store Read/1 -> Add/1
  Constant/1 -> Add/2
  "PDU_OUT "/1 -> Bus Selector1/1
  Bus Selector1/3 -> ?  "<VCU_ShrRlyCtl>"
  Bus Selector1/2 -> ?  "<VCU_HghVtgCtl>"
  Bus Selector1/1 -> ?  "<VCU_DCCpstRlyCtl>"
  Data Store Read1/1 -> Data Type Conversion/1
  Data Type Conversion/1 -> VCU_PDU/4
  Data Store Read6/1 -> Data Type Conversion1/1
  Data Type Conversion1/1 -> VCU_PDU/2
  Data Type Conversion2/1 -> VCU_PDU/5
  Data Store Read7/1 -> Data Type Conversion2/1
  Data Store Read5/1 -> Data Type Conversion3/1
  Data Type Conversion3/1 -> VCU_PDU/6
  Data Store Read8/1 -> Data Type Conversion4/1
  Data Type Conversion4/1 -> VCU_PDU/3
  Data Store Read9/1 -> Data Type Conversion5/1
  Data Type Conversion5/1 -> VCU_PDU/1

== system ZT_VehCtrl_18B_CAN/SigOut/TM ==
  "TM_OUT " : Inport
  Trigger : TriggerPort  VariantControl=Variant  PortDimensions=1
  Add : Sum
  Bus Selector : BusSelector  OutputSignals=Data,Length
  Constant : Constant  OutDataTypeStr=uint8
  Constant{1..10} (10 alike) : Constant  Value=0
  Data Store Read : DataStoreRead  DataStoreName=Cnt_TM_OUT
  Data Store Write : DataStoreWrite  DataStoreName=Cnt_TM_OUT
  FCAN_Send_ID_0xCFF05EF : mbd_mpc574x_ec_toolbox/Communication Blocks/CAN Blocks/FCAN_Send  Priority=2  can_instance=1  can_mode=Non-blocking  can_timeout_ms=0  can_mb_idx=53  can_extended_id=on  can_is_remote=off  can_id=CFF05EF  show_adv_opts=off  can_fd_enable=off  can_enable_brs=off  can_fd_padding=0
      settings: SourceProductName=NXP Model-Based Design Toolbox for MPC57xx MCUs
  TM HCU Command : canmsglib/CAN Pack  CANdbFile=D:\VCU\VCU_SL_ZhengZhou\ZT2\模型与接口\CAN_DBC\动力CANB_GBK.dbc  MsgList=(none)  MsgName=TM_HCU_Command  MsgIDType=Extended (29-bit identifier)  MsgIdentifier=218039791  MsgLength=8  SignalInfo=Control_Mode$2$2$1$2$1$0$1$0$-Inf$Inf$#Demand_Limit_High_Positive_Value$8$12$1$2$1$0$4$0$0$16384$#Demand_Limit_Low_Negative_Value$20$12$1$2$1$0$4$0$0$16384$#Demand_Speed$48$16$1$2$1$0$1$-15000$-15000$15000$#Demand_Torque$32$16$1$2$1$0$1$-5000$-5000$5000$#Fault_Reset$1$1$1$2$1$0$1$0$-Inf$Inf$#FootBrake$6$1$1$2$1$0$1$0$-Inf$Inf$#Gear$4$2$1$2$1$0$1$0$-Inf$Inf$#HandBrake$7$1$1$2$1$0$1$0$-Inf$Inf$#MCU_Enable$0$1$1$2$1$0$1$0$-Inf$Inf$#  NSignals=10  StartBits=str2num('[int32(2);int32(8);int32(20);int32(48);int32(32);int32(1);int32(6);int32(4);int32(7);int32(0)]')  SignalSizes=str2num('[int32(2);int32(12);int32(12);int32(16);int32(16);int32(1);int32(1);int32(2);int32(1);int32(1)]')  ByteOrders=str2num('[int32(1);int32(1);int32(1);int32(1);int32(1);int32(1);int32(1);int32(1);int32(1);int32(1)]')  DataTypes=str2num('[int32(2);int32(2);int32(2);int32(2);int32(2);int32(2);int32(2);int32(2);int32(2);int32(2)]')  MultiplexTypes=str2num('[int32(1);int32(1);int32(1);int32(1);int32(1);int32(1);int32(1);int32(1);int32(1);int32(1)]')  MultiplexValues=str2num('[double(0);double(0);double(0);double(0);double(0);double(0);double(0);double(0);double(0);double(0)]')  Factors=str2num('[double(1);double(4);double(4);double(1);double(1);double(1);double(1);double(1);double(1);double(1)]')  Offsets=str2num('[double(0);double(0);double(0);double(-15000);double(-5000);double(0);double(0);double(0);double(0);double(0)]')  Minimums=str2num('[double(-Inf);double(0);double(0);double(-15000);double(-5000);double(-Inf);double(-Inf);double(-Inf);double(-Inf);double(-Inf)]')  Maximums=str2num('[double(Inf);double(16384);double(16384);double(15000);double(5000);double(Inf);double(Inf);double(Inf);double(Inf);double(Inf)]')  Remote=off  ApplyMinMax=off  BusOutput=on
      settings: SourceProductName=Simulink Real-Time  SourceProductBaseCode=XP  DataFormat=CANdb specified signals
  Terminator : Terminator
  wires:
  Bus Selector/1 -> FCAN_Send_ID_0xCFF05EF/1  "<Data>"
  Bus Selector/2 -> FCAN_Send_ID_0xCFF05EF/2  "<Length>"
  TM HCU Command/1 -> Bus Selector/1
  "TM_OUT "/1 -> Terminator/1
  Constant1/1 -> TM HCU Command/1
  Constant2/1 -> TM HCU Command/2
  Constant3/1 -> TM HCU Command/3
  Constant4/1 -> TM HCU Command/4
  Constant5/1 -> TM HCU Command/5
  Constant6/1 -> TM HCU Command/6
  Constant7/1 -> TM HCU Command/7
  Constant8/1 -> TM HCU Command/8
  Constant9/1 -> TM HCU Command/9
  Constant10/1 -> TM HCU Command/10
  Add/1 -> Data Store Write/1
  Data Store Read/1 -> Add/1
  Constant/1 -> Add/2

== system ZT_VehCtrl_18B_CAN/SigOut/TMS ==
  "TMS_OUT " : Inport
  Trigger : TriggerPort  VariantControl=Variant  PortDimensions=1
  Add : Sum
  Bus Selector : BusSelector  OutputSignals=Data,Length
  Bus Selector2 : BusSelector  Commented=on  OutputSignals=signal6.AccPadle,BMS.VCU_BattBusCurr_A
  Constant : Constant  OutDataTypeStr=uint8
  Data Store Read : DataStoreRead  DataStoreName=Cnt_TMS_OUT
  Data Store Read1 : DataStoreRead  DataStoreName=Cnt_TMS_OUT
  Data Store Read3 : DataStoreRead  DataStoreName=VCU_FanSpeedLvl_num
  Data Store Write : DataStoreWrite  DataStoreName=Cnt_TMS_OUT
  Data Type Conversion : DataTypeConversion
  FCAN_Send_ID_0x18FFF347 : mbd_mpc574x_ec_toolbox/Communication Blocks/CAN Blocks/FCAN_Send  Priority=2  can_instance=0  can_mode=Non-blocking  can_timeout_ms=0  can_mb_idx=15  can_extended_id=on  can_is_remote=off  can_id=18FFF347  show_adv_opts=off  can_fd_enable=off  can_enable_brs=off  can_fd_padding=0
      settings: SourceProductName=NXP Model-Based Design Toolbox for MPC57xx MCUs
  TMS : canmsglib/CAN Pack  CANdbFile=D:\VCU\VCU_SL_ZhengZhou\ZT2\模型与接口\CAN_DBC\整车CANA_GBK.dbc  MsgList=(none)  MsgName=VCU2TMS  MsgIDType=Extended (29-bit identifier)  MsgIdentifier=419427143  MsgLength=8  SignalInfo=VCU_FanSpeedLvl_num$0$8$2$2$1$0$1$0$0$255$#VCU_Life1_num$56$8$2$2$1$0$1$0$0$255$#  NSignals=2  StartBits=str2num('[int32(0);int32(56)]')  SignalSizes=str2num('[int32(8);int32(8)]')  ByteOrders=str2num('[int32(2);int32(2)]')  DataTypes=str2num('[int32(2);int32(2)]')  MultiplexTypes=str2num('[int32(1);int32(1)]')  MultiplexValues=str2num('[double(0);double(0)]')  Factors=str2num('[double(1);double(1)]')  Offsets=str2num('[double(0);double(0)]')  Minimums=str2num('[double(0);double(0)]')  Maximums=str2num('[double(255);double(255)]')  Remote=off  ApplyMinMax=off  BusOutput=on
      settings: SourceProductName=Simulink Real-Time  SourceProductBaseCode=XP  DataFormat=CANdb specified signals
  wires:
  TMS/1 -> Bus Selector/1
  Bus Selector/1 -> FCAN_Send_ID_0x18FFF347/1  "<Data>"
  Bus Selector/2 -> FCAN_Send_ID_0x18FFF347/2  "<Length>"
  Add/1 -> Data Store Write/1
  Data Store Read/1 -> Add/1
  Constant/1 -> Add/2
  "TMS_OUT "/1 -> Bus Selector2/1
  Data Store Read3/1 -> Data Type Conversion/1
  Data Type Conversion/1 -> TMS/1
  Data Store Read1/1 -> TMS/2

== system ZT_VehCtrl_18B_CAN/SigOut/TWV ==
  "TWV_OUT " : Inport
  Trigger : TriggerPort  VariantControl=Variant  PortDimensions=1
  Add : Sum
  Bus Selector : BusSelector  OutputSignals=Data,Length
  Bus Selector1 : BusSelector  Commented=on  OutputSignals=signal1,signal2
  Constant : Constant  OutDataTypeStr=uint8
  Data Store Read : DataStoreRead  DataStoreName=Cnt_TWV_OUT
  Data Store Read10 : DataStoreRead  DataStoreName=TWV_ON_Ctr
  Data Store Write : DataStoreWrite  DataStoreName=Cnt_TWV_OUT
  Data Type Conversion : DataTypeConversion  OutDataTypeStr=single
  FCAN_Send_ID_0x18FF25EF : mbd_mpc574x_ec_toolbox/Communication Blocks/CAN Blocks/FCAN_Send  Priority=2  can_instance=1  can_mode=Non-blocking  can_timeout_ms=0  can_mb_idx=55  can_extended_id=on  can_is_remote=off  can_id=0  show_adv_opts=off  can_fd_enable=off  can_enable_brs=off  can_fd_padding=0
      settings: SourceProductName=NXP Model-Based Design Toolbox for MPC57xx MCUs
  VCU_TWV : canmsglib/CAN Pack  CANdbFile=D:\VCU\VCU_SL_ZhengZhou\ZT2\Module\CAN_DBC\所有CAN信号\动力CAN.dbc  MsgList=VCU_TWV  MsgName=VCU_TWV  MsgIDType=Extended (29-bit identifier)  MsgIdentifier=217933600  MsgLength=8  SignalInfo=TWV_ON_Ctr$0$7$1$2$1$0$1$0$0$127$#  NSignals=1  StartBits=str2num('[int32(0)]')  SignalSizes=str2num('[int32(7)]')  ByteOrders=str2num('[int32(1)]')  DataTypes=str2num('[int32(2)]')  MultiplexTypes=str2num('[int32(1)]')  MultiplexValues=str2num('[double(0)]')  Factors=str2num('[double(1)]')  Offsets=str2num('[double(0)]')  Minimums=str2num('[double(0)]')  Maximums=str2num('[double(127)]')  Remote=off  ApplyMinMax=off  BusOutput=on
      settings: SourceProductName=Simulink Real-Time  SourceProductBaseCode=XP  DataFormat=CANdb specified signals
  wires:
  VCU_TWV/1 -> Bus Selector/1
  Bus Selector/2 -> FCAN_Send_ID_0x18FF25EF/2  "<Length>"
  Bus Selector/1 -> FCAN_Send_ID_0x18FF25EF/1  "<Data>"
  Add/1 -> Data Store Write/1
  Data Store Read/1 -> Add/1
  Constant/1 -> Add/2
  Data Store Read10/1 -> Data Type Conversion/1
  Data Type Conversion/1 -> VCU_TWV/1
  "TWV_OUT "/1 -> Bus Selector1/1
